simulink model "models_confrontation"  (R2023b)
settings: Solver=VariableStepAuto  StartTime=0.0  StopTime=150  RelTol=1e-3
values from neighbouring files (symbols this model uses):
  A_disc = [0.952255240734 0.0558764138291 0.00101235520744 -0.119343099159 -0.00359337854643 0.0465636781909 0.897600307888 0.0332309130595 0.226714958367 0.0683979085849 0.00118108107535 0.0465232782833 ... (25 elements, 5x5)]    [linear_model.mat]    (also in tank_confrontation_init.m = sys_disc.A)
  B_disc = [0 0 0 0.228023543382 0.0100072301308 0.406395598078 0.00344423879117 -0.350799254632 -0.030419989559 0.036993899484 -0.000142908764649 -0.00850948072699 ... (15 elements, 5x3)]    [linear_model.mat]    (also in tank_confrontation_init.m = sys_disc.B)
  c2_init = c2_0    [tank_confrontation_init.m]
  c3_init = c3_0    [tank_confrontation_init.m]
  C_disc = [0 0 0 1 0 0 0 1 0 0 0 0 ... (15 elements, 3x5)]    [linear_model.mat]    (also in tank_confrontation_init.m = sys_disc.C)
  D_disc = [0  0  0; 0  0  0; 0  0  0]    [linear_model.mat]    (also in tank_confrontation_init.m = sys_disc.D)
  h1_init = h1_0    [tank_confrontation_init.m]
  h2_init = h2_0    [tank_confrontation_init.m]
  h3_init = h3_0    [tank_confrontation_init.m]
  sample_time = 2.0    (= 2)    [tank_confrontation_init.m]
  u_star = [1.78740880431 0.02 0.18]    [linear_model.mat]
  y_star = [x_star(2); x_star(3); x_star(5)]    [tank_confrontation_init.m]
undefined symbols (not defined in the file or in its folder): DiscIntNeverNeededParam, params
libraries: slpidlib x9
settings Model: Creator=fyder9  LastModifiedBy=fyder9

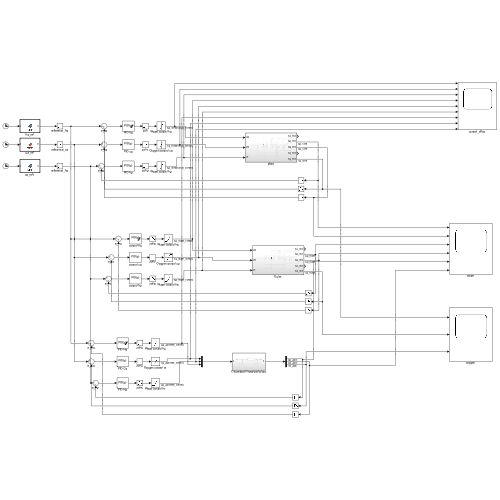
[thumbnail: Simulink's stored preview of the top-level diagram]
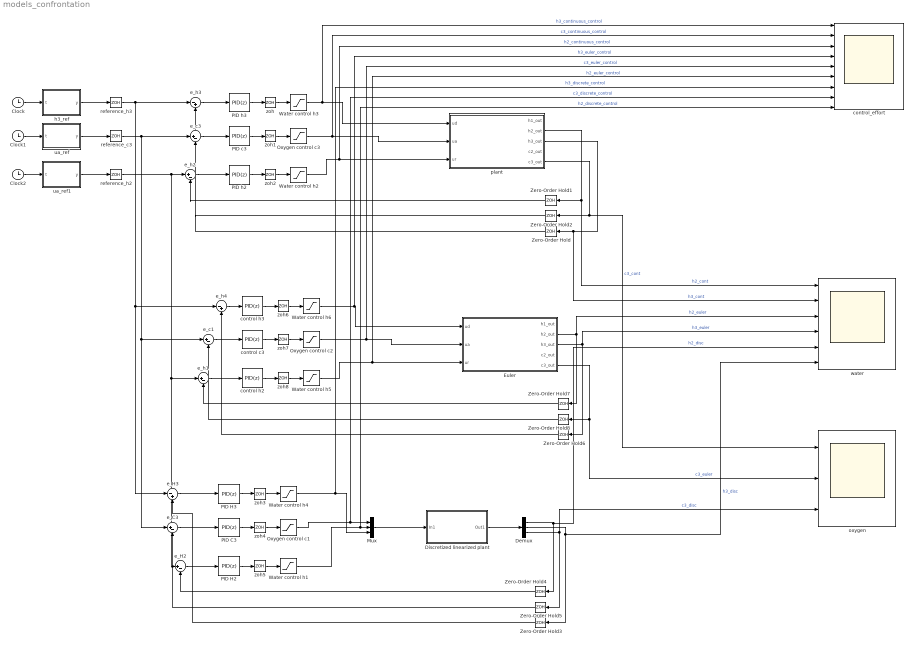
== system models_confrontation ==
  Clock : Clock
  Clock1 : Clock
  Clock2 : Clock
  Demux : Demux  Outputs=3
  Discretized linearized plant : Subsystem
  Euler : Subsystem
  Mux : Mux  Inputs=3
  Oxygen control c1 : Saturate  UpperLimit=1  LowerLimit=0  LinearizeAsGain=off
  Oxygen control c2 : Saturate  UpperLimit=1  LowerLimit=0  LinearizeAsGain=off
  Oxygen control c3 : Saturate  UpperLimit=1  LowerLimit=0  LinearizeAsGain=off
  PID C3 : slpidlib/PID Controller  Controller=PID  Form=Parallel  TimeDomain=Discrete-time  UseExternalTs=off  SampleTime=-1  IntegratorMethod=Forward Euler  FilterMethod=Forward Euler  ControllerParametersSource=internal  P=0.1  I=0.02  UseKiTs=off  D=0  N=100  UseFilter=on  TunerSelectOption=Transfer Function Based (PID Tuner App)  InitialConditionSource=internal  InitialConditionForIntegrator=0  InitialConditionForFilter=0  DifferentiatorICPrevScaledInput=0  ExternalReset=none  TrackingMode=off  Kt=1  LimitOutput=off  SatLimitsSource=internal  UpperSaturationLimit=inf  LowerSaturationLimit=-inf  LinearizeAsGain=off  AntiWindupMode=none  Kb=1  LimitIntegrator=off  UpperIntegratorSaturationLimit=inf  LowerIntegratorSaturationLimit=-inf  POutMin=[]  POutMax=[]  IOutMin=[]  IOutMax=[]  DOutMin=[]  DOutMax=[]  NOutMin=[]  NOutMax=[]  SumOutMin=[]  SumOutMax=[]  SaturationOutMin=[]  SaturationOutMax=[]  PParamMin=[]  PParamMax=[]  IParamMin=[]  IParamMax=[]  DParamMin=[]  DParamMax=[]  NParamMin=[]  NParamMax=[]  KbParamMin=[]  KbParamMax=[]  KtParamMin=[]  KtParamMax=[]  KbOutMin=[]  KbOutMax=[]  KtOutMin=[]  KtOutMax=[]  IntegratorOutMin=[]  IntegratorOutMax=[]  FilterOutMin=[]  FilterOutMax=[]  SumI1OutMin=[]  SumI1OutMax=[]  SumI2OutMin=[]  SumI2OutMax=[]  SumI3OutMin=[]  SumI3OutMax=[]  SumI4OutMin=[]  SumI4OutMax=[]  SumDOutMin=[]  SumDOutMax=[]  DifferentiatorOutMin=[]  DifferentiatorOutMax=[]  FilterDiffOutCoefMin=[]  FilterDiffOutCoefMax=[]  ReciprocalOutMin=[]  ReciprocalOutMax=[]  SumDenOutMin=[]  SumDenOutMax=[]  SumNumOutMin=[]  SumNumOutMax=[]  DivideOutMin=[]  DivideOutMax=[]  UdiffTsProdOutMin=[]  UdiffTsProdOutMax=[]  NTsProdOutMin=[]  NTsProdOutMax=[]  UintegralTsProdOutMin=[]  UintegralTsProdOutMax=[]  UngainTsProdOutMin=[]  UngainTsProdOutMax=[]  ClampingZeroOutDataTypeStr=Inherit: Inherit via back propagation  ClampingZeroOutMin=[]  ClampingZeroOutMax=[]  FilterDenConstantOutDataTypeStr=Inherit: Inherit via back propagation  FilterDenConstantOutMin=[]  FilterDenConstantOutMax=[]  PCopyOutDataTypeStr=Inherit: Inherit via back propagation  PCopyOutMin=[]  PCopyOutMax=[]  NCopyOutDataTypeStr=Inherit: Inherit via back propagation  NCopyOutMin=[]  NCopyOutMax=[]  IntegratorContinuousStateAttributes=''  IntegratorStateMustResolveToSignalObject=off  IntegratorRTWStateStorageClass=Auto  FilterContinuousStateAttributes=''  FilterStateMustResolveToSignalObject=off  FilterRTWStateStorageClass=Auto  ParallelPVariant=InternalParameters  IdealPVariant=Disabled  IVariant=InternalParameters  DVariant=InternalParameters  IntegratorVariant=Discrete  SatVariant=Disabled  AWVariant=Passthrough  PCopyVariant=Disabled  TRVariant=Disabled  FdbkBlocksVariant=Forward  IdealPFdbkVariant=Disabled  SatFdbkVariant=Disabled  DerivativeFilterVariant=ForwardEulerFilter  NVariant=InternalParameters  NCopyVariant=Disabled  FilterICVariant=InternalICsFilter  IntegratorICVariant=InternalICs  ExternalResetVariant=Disabled  TRSumVariant=Passthrough  SumFdbkVariant=Disabled  SumVariant=Sum_PID  TsampFilterVariant=InternalTs  TsampNgainVariant=Passthrough  TsampIntegralVariant=Disabled_SignalSpec  ExternalSaturationOutDataTypeStr=Inherit: Same as second input
      settings: LibrarySourceBlock=simulink/Discrete/Discrete PID Controller
  PID H2 : slpidlib/PID Controller  Controller=PID  Form=Parallel  TimeDomain=Discrete-time  UseExternalTs=off  SampleTime=-1  IntegratorMethod=Forward Euler  FilterMethod=Forward Euler  ControllerParametersSource=internal  P=0.2  I=0.03  UseKiTs=off  D=0  N=100  UseFilter=on  TunerSelectOption=Transfer Function Based (PID Tuner App)  InitialConditionSource=internal  InitialConditionForIntegrator=0  InitialConditionForFilter=0  DifferentiatorICPrevScaledInput=0  ExternalReset=none  TrackingMode=off  Kt=1  LimitOutput=off  SatLimitsSource=internal  UpperSaturationLimit=inf  LowerSaturationLimit=-inf  LinearizeAsGain=off  AntiWindupMode=none  Kb=1  LimitIntegrator=off  UpperIntegratorSaturationLimit=inf  LowerIntegratorSaturationLimit=-inf  POutMin=[]  POutMax=[]  IOutMin=[]  IOutMax=[]  DOutMin=[]  DOutMax=[]  NOutMin=[]  NOutMax=[]  SumOutMin=[]  SumOutMax=[]  SaturationOutMin=[]  SaturationOutMax=[]  PParamMin=[]  PParamMax=[]  IParamMin=[]  IParamMax=[]  DParamMin=[]  DParamMax=[]  NParamMin=[]  NParamMax=[]  KbParamMin=[]  KbParamMax=[]  KtParamMin=[]  KtParamMax=[]  KbOutMin=[]  KbOutMax=[]  KtOutMin=[]  KtOutMax=[]  IntegratorOutMin=[]  IntegratorOutMax=[]  FilterOutMin=[]  FilterOutMax=[]  SumI1OutMin=[]  SumI1OutMax=[]  SumI2OutMin=[]  SumI2OutMax=[]  SumI3OutMin=[]  SumI3OutMax=[]  SumI4OutMin=[]  SumI4OutMax=[]  SumDOutMin=[]  SumDOutMax=[]  DifferentiatorOutMin=[]  DifferentiatorOutMax=[]  FilterDiffOutCoefMin=[]  FilterDiffOutCoefMax=[]  ReciprocalOutMin=[]  ReciprocalOutMax=[]  SumDenOutMin=[]  SumDenOutMax=[]  SumNumOutMin=[]  SumNumOutMax=[]  DivideOutMin=[]  DivideOutMax=[]  UdiffTsProdOutMin=[]  UdiffTsProdOutMax=[]  NTsProdOutMin=[]  NTsProdOutMax=[]  UintegralTsProdOutMin=[]  UintegralTsProdOutMax=[]  UngainTsProdOutMin=[]  UngainTsProdOutMax=[]  ClampingZeroOutDataTypeStr=Inherit: Inherit via back propagation  ClampingZeroOutMin=[]  ClampingZeroOutMax=[]  FilterDenConstantOutDataTypeStr=Inherit: Inherit via back propagation  FilterDenConstantOutMin=[]  FilterDenConstantOutMax=[]  PCopyOutDataTypeStr=Inherit: Inherit via back propagation  PCopyOutMin=[]  PCopyOutMax=[]  NCopyOutDataTypeStr=Inherit: Inherit via back propagation  NCopyOutMin=[]  NCopyOutMax=[]  IntegratorContinuousStateAttributes=''  IntegratorStateMustResolveToSignalObject=off  IntegratorRTWStateStorageClass=Auto  FilterContinuousStateAttributes=''  FilterStateMustResolveToSignalObject=off  FilterRTWStateStorageClass=Auto  ParallelPVariant=InternalParameters  IdealPVariant=Disabled  IVariant=InternalParameters  DVariant=InternalParameters  IntegratorVariant=Discrete  SatVariant=Disabled  AWVariant=Passthrough  PCopyVariant=Disabled  TRVariant=Disabled  FdbkBlocksVariant=Forward  IdealPFdbkVariant=Disabled  SatFdbkVariant=Disabled  DerivativeFilterVariant=ForwardEulerFilter  NVariant=InternalParameters  NCopyVariant=Disabled  FilterICVariant=InternalICsFilter  IntegratorICVariant=InternalICs  ExternalResetVariant=Disabled  TRSumVariant=Passthrough  SumFdbkVariant=Disabled  SumVariant=Sum_PID  TsampFilterVariant=InternalTs  TsampNgainVariant=Passthrough  TsampIntegralVariant=Disabled_SignalSpec  ExternalSaturationOutDataTypeStr=Inherit: Same as second input
      settings: LibrarySourceBlock=simulink/Discrete/Discrete PID Controller
  PID H3 : slpidlib/PID Controller  Controller=PID  Form=Parallel  TimeDomain=Discrete-time  UseExternalTs=off  SampleTime=-1  IntegratorMethod=Forward Euler  FilterMethod=Forward Euler  ControllerParametersSource=internal  P=0.6  I=0.08  UseKiTs=off  D=0  N=100  UseFilter=on  TunerSelectOption=Transfer Function Based (PID Tuner App)  InitialConditionSource=internal  InitialConditionForIntegrator=0  InitialConditionForFilter=0  DifferentiatorICPrevScaledInput=0  ExternalReset=none  TrackingMode=off  Kt=1  LimitOutput=on  SatLimitsSource=internal  UpperSaturationLimit=inf  LowerSaturationLimit=-inf  LinearizeAsGain=off  AntiWindupMode=clamping  Kb=1  LimitIntegrator=off  UpperIntegratorSaturationLimit=inf  LowerIntegratorSaturationLimit=-inf  POutMin=[]  POutMax=[]  IOutMin=[]  IOutMax=[]  DOutMin=[]  DOutMax=[]  NOutMin=[]  NOutMax=[]  SumOutMin=[]  SumOutMax=[]  SaturationOutMin=[]  SaturationOutMax=[]  PParamMin=[]  PParamMax=[]  IParamMin=[]  IParamMax=[]  DParamMin=[]  DParamMax=[]  NParamMin=[]  NParamMax=[]  KbParamMin=[]  KbParamMax=[]  KtParamMin=[]  KtParamMax=[]  KbOutMin=[]  KbOutMax=[]  KtOutMin=[]  KtOutMax=[]  IntegratorOutMin=[]  IntegratorOutMax=[]  FilterOutMin=[]  FilterOutMax=[]  SumI1OutMin=[]  SumI1OutMax=[]  SumI2OutMin=[]  SumI2OutMax=[]  SumI3OutMin=[]  SumI3OutMax=[]  SumI4OutMin=[]  SumI4OutMax=[]  SumDOutMin=[]  SumDOutMax=[]  DifferentiatorOutMin=[]  DifferentiatorOutMax=[]  FilterDiffOutCoefMin=[]  FilterDiffOutCoefMax=[]  ReciprocalOutMin=[]  ReciprocalOutMax=[]  SumDenOutMin=[]  SumDenOutMax=[]  SumNumOutMin=[]  SumNumOutMax=[]  DivideOutMin=[]  DivideOutMax=[]  UdiffTsProdOutMin=[]  UdiffTsProdOutMax=[]  NTsProdOutMin=[]  NTsProdOutMax=[]  UintegralTsProdOutMin=[]  UintegralTsProdOutMax=[]  UngainTsProdOutMin=[]  UngainTsProdOutMax=[]  ClampingZeroOutDataTypeStr=Inherit: Inherit via back propagation  ClampingZeroOutMin=[]  ClampingZeroOutMax=[]  FilterDenConstantOutDataTypeStr=Inherit: Inherit via back propagation  FilterDenConstantOutMin=[]  FilterDenConstantOutMax=[]  PCopyOutDataTypeStr=Inherit: Inherit via back propagation  PCopyOutMin=[]  PCopyOutMax=[]  NCopyOutDataTypeStr=Inherit: Inherit via back propagation  NCopyOutMin=[]  NCopyOutMax=[]  IntegratorContinuousStateAttributes=''  IntegratorStateMustResolveToSignalObject=off  IntegratorRTWStateStorageClass=Auto  FilterContinuousStateAttributes=''  FilterStateMustResolveToSignalObject=off  FilterRTWStateStorageClass=Auto  ParallelPVariant=InternalParameters  IdealPVariant=Disabled  IVariant=InternalParameters  DVariant=InternalParameters  IntegratorVariant=Discrete  SatVariant=Enabled  AWVariant=DiscClampingParallel  PCopyVariant=Disabled  TRVariant=Disabled  FdbkBlocksVariant=Forward  IdealPFdbkVariant=Disabled  SatFdbkVariant=Disabled  DerivativeFilterVariant=ForwardEulerFilter  NVariant=InternalParameters  NCopyVariant=Disabled  FilterICVariant=InternalICsFilter  IntegratorICVariant=InternalICs  ExternalResetVariant=Disabled  TRSumVariant=Passthrough  SumFdbkVariant=Disabled  SumVariant=Sum_PID  TsampFilterVariant=InternalTs  TsampNgainVariant=Passthrough  TsampIntegralVariant=Disabled_SignalSpec  ExternalSaturationOutDataTypeStr=Inherit: Same as second input
      settings: LibrarySourceBlock=simulink/Discrete/Discrete PID Controller
  PID c3 : slpidlib/PID Controller  Controller=PID  Form=Parallel  TimeDomain=Discrete-time  UseExternalTs=off  SampleTime=-1  IntegratorMethod=Forward Euler  FilterMethod=Forward Euler  ControllerParametersSource=internal  P=0.1  I=0.02  UseKiTs=off  D=0  N=100  UseFilter=on  TunerSelectOption=Transfer Function Based (PID Tuner App)  InitialConditionSource=internal  InitialConditionForIntegrator=0  InitialConditionForFilter=0  DifferentiatorICPrevScaledInput=0  ExternalReset=none  TrackingMode=off  Kt=1  LimitOutput=off  SatLimitsSource=internal  UpperSaturationLimit=inf  LowerSaturationLimit=-inf  LinearizeAsGain=off  AntiWindupMode=none  Kb=1  LimitIntegrator=off  UpperIntegratorSaturationLimit=inf  LowerIntegratorSaturationLimit=-inf  POutMin=[]  POutMax=[]  IOutMin=[]  IOutMax=[]  DOutMin=[]  DOutMax=[]  NOutMin=[]  NOutMax=[]  SumOutMin=[]  SumOutMax=[]  SaturationOutMin=[]  SaturationOutMax=[]  PParamMin=[]  PParamMax=[]  IParamMin=[]  IParamMax=[]  DParamMin=[]  DParamMax=[]  NParamMin=[]  NParamMax=[]  KbParamMin=[]  KbParamMax=[]  KtParamMin=[]  KtParamMax=[]  KbOutMin=[]  KbOutMax=[]  KtOutMin=[]  KtOutMax=[]  IntegratorOutMin=[]  IntegratorOutMax=[]  FilterOutMin=[]  FilterOutMax=[]  SumI1OutMin=[]  SumI1OutMax=[]  SumI2OutMin=[]  SumI2OutMax=[]  SumI3OutMin=[]  SumI3OutMax=[]  SumI4OutMin=[]  SumI4OutMax=[]  SumDOutMin=[]  SumDOutMax=[]  DifferentiatorOutMin=[]  DifferentiatorOutMax=[]  FilterDiffOutCoefMin=[]  FilterDiffOutCoefMax=[]  ReciprocalOutMin=[]  ReciprocalOutMax=[]  SumDenOutMin=[]  SumDenOutMax=[]  SumNumOutMin=[]  SumNumOutMax=[]  DivideOutMin=[]  DivideOutMax=[]  UdiffTsProdOutMin=[]  UdiffTsProdOutMax=[]  NTsProdOutMin=[]  NTsProdOutMax=[]  UintegralTsProdOutMin=[]  UintegralTsProdOutMax=[]  UngainTsProdOutMin=[]  UngainTsProdOutMax=[]  ClampingZeroOutDataTypeStr=Inherit: Inherit via back propagation  ClampingZeroOutMin=[]  ClampingZeroOutMax=[]  FilterDenConstantOutDataTypeStr=Inherit: Inherit via back propagation  FilterDenConstantOutMin=[]  FilterDenConstantOutMax=[]  PCopyOutDataTypeStr=Inherit: Inherit via back propagation  PCopyOutMin=[]  PCopyOutMax=[]  NCopyOutDataTypeStr=Inherit: Inherit via back propagation  NCopyOutMin=[]  NCopyOutMax=[]  IntegratorContinuousStateAttributes=''  IntegratorStateMustResolveToSignalObject=off  IntegratorRTWStateStorageClass=Auto  FilterContinuousStateAttributes=''  FilterStateMustResolveToSignalObject=off  FilterRTWStateStorageClass=Auto  ParallelPVariant=InternalParameters  IdealPVariant=Disabled  IVariant=InternalParameters  DVariant=InternalParameters  IntegratorVariant=Discrete  SatVariant=Disabled  AWVariant=Passthrough  PCopyVariant=Disabled  TRVariant=Disabled  FdbkBlocksVariant=Forward  IdealPFdbkVariant=Disabled  SatFdbkVariant=Disabled  DerivativeFilterVariant=ForwardEulerFilter  NVariant=InternalParameters  NCopyVariant=Disabled  FilterICVariant=InternalICsFilter  IntegratorICVariant=InternalICs  ExternalResetVariant=Disabled  TRSumVariant=Passthrough  SumFdbkVariant=Disabled  SumVariant=Sum_PID  TsampFilterVariant=InternalTs  TsampNgainVariant=Passthrough  TsampIntegralVariant=Disabled_SignalSpec  ExternalSaturationOutDataTypeStr=Inherit: Same as second input
      settings: LibrarySourceBlock=simulink/Discrete/Discrete PID Controller
  PID h2 : slpidlib/PID Controller  Controller=PID  Form=Parallel  TimeDomain=Discrete-time  UseExternalTs=off  SampleTime=-1  IntegratorMethod=Forward Euler  FilterMethod=Forward Euler  ControllerParametersSource=internal  P=0.2  I=0.03  UseKiTs=off  D=0  N=100  UseFilter=on  TunerSelectOption=Transfer Function Based (PID Tuner App)  InitialConditionSource=internal  InitialConditionForIntegrator=0  InitialConditionForFilter=0  DifferentiatorICPrevScaledInput=0  ExternalReset=none  TrackingMode=off  Kt=1  LimitOutput=off  SatLimitsSource=internal  UpperSaturationLimit=inf  LowerSaturationLimit=-inf  LinearizeAsGain=off  AntiWindupMode=none  Kb=1  LimitIntegrator=off  UpperIntegratorSaturationLimit=inf  LowerIntegratorSaturationLimit=-inf  POutMin=[]  POutMax=[]  IOutMin=[]  IOutMax=[]  DOutMin=[]  DOutMax=[]  NOutMin=[]  NOutMax=[]  SumOutMin=[]  SumOutMax=[]  SaturationOutMin=[]  SaturationOutMax=[]  PParamMin=[]  PParamMax=[]  IParamMin=[]  IParamMax=[]  DParamMin=[]  DParamMax=[]  NParamMin=[]  NParamMax=[]  KbParamMin=[]  KbParamMax=[]  KtParamMin=[]  KtParamMax=[]  KbOutMin=[]  KbOutMax=[]  KtOutMin=[]  KtOutMax=[]  IntegratorOutMin=[]  IntegratorOutMax=[]  FilterOutMin=[]  FilterOutMax=[]  SumI1OutMin=[]  SumI1OutMax=[]  SumI2OutMin=[]  SumI2OutMax=[]  SumI3OutMin=[]  SumI3OutMax=[]  SumI4OutMin=[]  SumI4OutMax=[]  SumDOutMin=[]  SumDOutMax=[]  DifferentiatorOutMin=[]  DifferentiatorOutMax=[]  FilterDiffOutCoefMin=[]  FilterDiffOutCoefMax=[]  ReciprocalOutMin=[]  ReciprocalOutMax=[]  SumDenOutMin=[]  SumDenOutMax=[]  SumNumOutMin=[]  SumNumOutMax=[]  DivideOutMin=[]  DivideOutMax=[]  UdiffTsProdOutMin=[]  UdiffTsProdOutMax=[]  NTsProdOutMin=[]  NTsProdOutMax=[]  UintegralTsProdOutMin=[]  UintegralTsProdOutMax=[]  UngainTsProdOutMin=[]  UngainTsProdOutMax=[]  ClampingZeroOutDataTypeStr=Inherit: Inherit via back propagation  ClampingZeroOutMin=[]  ClampingZeroOutMax=[]  FilterDenConstantOutDataTypeStr=Inherit: Inherit via back propagation  FilterDenConstantOutMin=[]  FilterDenConstantOutMax=[]  PCopyOutDataTypeStr=Inherit: Inherit via back propagation  PCopyOutMin=[]  PCopyOutMax=[]  NCopyOutDataTypeStr=Inherit: Inherit via back propagation  NCopyOutMin=[]  NCopyOutMax=[]  IntegratorContinuousStateAttributes=''  IntegratorStateMustResolveToSignalObject=off  IntegratorRTWStateStorageClass=Auto  FilterContinuousStateAttributes=''  FilterStateMustResolveToSignalObject=off  FilterRTWStateStorageClass=Auto  ParallelPVariant=InternalParameters  IdealPVariant=Disabled  IVariant=InternalParameters  DVariant=InternalParameters  IntegratorVariant=Discrete  SatVariant=Disabled  AWVariant=Passthrough  PCopyVariant=Disabled  TRVariant=Disabled  FdbkBlocksVariant=Forward  IdealPFdbkVariant=Disabled  SatFdbkVariant=Disabled  DerivativeFilterVariant=ForwardEulerFilter  NVariant=InternalParameters  NCopyVariant=Disabled  FilterICVariant=InternalICsFilter  IntegratorICVariant=InternalICs  ExternalResetVariant=Disabled  TRSumVariant=Passthrough  SumFdbkVariant=Disabled  SumVariant=Sum_PID  TsampFilterVariant=InternalTs  TsampNgainVariant=Passthrough  TsampIntegralVariant=Disabled_SignalSpec  ExternalSaturationOutDataTypeStr=Inherit: Same as second input
      settings: LibrarySourceBlock=simulink/Discrete/Discrete PID Controller
  PID h3 : slpidlib/PID Controller  Controller=PID  Form=Parallel  TimeDomain=Discrete-time  UseExternalTs=off  SampleTime=-1  IntegratorMethod=Forward Euler  FilterMethod=Forward Euler  ControllerParametersSource=internal  P=0.6  I=0.08  UseKiTs=off  D=0  N=100  UseFilter=on  TunerSelectOption=Transfer Function Based (PID Tuner App)  InitialConditionSource=internal  InitialConditionForIntegrator=0  InitialConditionForFilter=0  DifferentiatorICPrevScaledInput=0  ExternalReset=none  TrackingMode=off  Kt=1  LimitOutput=on  SatLimitsSource=internal  UpperSaturationLimit=inf  LowerSaturationLimit=-inf  LinearizeAsGain=off  AntiWindupMode=clamping  Kb=1  LimitIntegrator=off  UpperIntegratorSaturationLimit=inf  LowerIntegratorSaturationLimit=-inf  POutMin=[]  POutMax=[]  IOutMin=[]  IOutMax=[]  DOutMin=[]  DOutMax=[]  NOutMin=[]  NOutMax=[]  SumOutMin=[]  SumOutMax=[]  SaturationOutMin=[]  SaturationOutMax=[]  PParamMin=[]  PParamMax=[]  IParamMin=[]  IParamMax=[]  DParamMin=[]  DParamMax=[]  NParamMin=[]  NParamMax=[]  KbParamMin=[]  KbParamMax=[]  KtParamMin=[]  KtParamMax=[]  KbOutMin=[]  KbOutMax=[]  KtOutMin=[]  KtOutMax=[]  IntegratorOutMin=[]  IntegratorOutMax=[]  FilterOutMin=[]  FilterOutMax=[]  SumI1OutMin=[]  SumI1OutMax=[]  SumI2OutMin=[]  SumI2OutMax=[]  SumI3OutMin=[]  SumI3OutMax=[]  SumI4OutMin=[]  SumI4OutMax=[]  SumDOutMin=[]  SumDOutMax=[]  DifferentiatorOutMin=[]  DifferentiatorOutMax=[]  FilterDiffOutCoefMin=[]  FilterDiffOutCoefMax=[]  ReciprocalOutMin=[]  ReciprocalOutMax=[]  SumDenOutMin=[]  SumDenOutMax=[]  SumNumOutMin=[]  SumNumOutMax=[]  DivideOutMin=[]  DivideOutMax=[]  UdiffTsProdOutMin=[]  UdiffTsProdOutMax=[]  NTsProdOutMin=[]  NTsProdOutMax=[]  UintegralTsProdOutMin=[]  UintegralTsProdOutMax=[]  UngainTsProdOutMin=[]  UngainTsProdOutMax=[]  ClampingZeroOutDataTypeStr=Inherit: Inherit via back propagation  ClampingZeroOutMin=[]  ClampingZeroOutMax=[]  FilterDenConstantOutDataTypeStr=Inherit: Inherit via back propagation  FilterDenConstantOutMin=[]  FilterDenConstantOutMax=[]  PCopyOutDataTypeStr=Inherit: Inherit via back propagation  PCopyOutMin=[]  PCopyOutMax=[]  NCopyOutDataTypeStr=Inherit: Inherit via back propagation  NCopyOutMin=[]  NCopyOutMax=[]  IntegratorContinuousStateAttributes=''  IntegratorStateMustResolveToSignalObject=off  IntegratorRTWStateStorageClass=Auto  FilterContinuousStateAttributes=''  FilterStateMustResolveToSignalObject=off  FilterRTWStateStorageClass=Auto  ParallelPVariant=InternalParameters  IdealPVariant=Disabled  IVariant=InternalParameters  DVariant=InternalParameters  IntegratorVariant=Discrete  SatVariant=Enabled  AWVariant=DiscClampingParallel  PCopyVariant=Disabled  TRVariant=Disabled  FdbkBlocksVariant=Forward  IdealPFdbkVariant=Disabled  SatFdbkVariant=Disabled  DerivativeFilterVariant=ForwardEulerFilter  NVariant=InternalParameters  NCopyVariant=Disabled  FilterICVariant=InternalICsFilter  IntegratorICVariant=InternalICs  ExternalResetVariant=Disabled  TRSumVariant=Passthrough  SumFdbkVariant=Disabled  SumVariant=Sum_PID  TsampFilterVariant=InternalTs  TsampNgainVariant=Passthrough  TsampIntegralVariant=Disabled_SignalSpec  ExternalSaturationOutDataTypeStr=Inherit: Same as second input
      settings: LibrarySourceBlock=simulink/Discrete/Discrete PID Controller
  Water control h{1..6} (6 alike) : Saturate  UpperLimit=0.25  LowerLimit=0.05  LinearizeAsGain=off
  Zero-Order Hold{,1..8} (9 alike) : ZeroOrderHold  SampleTime=sample_time
  control c3 : slpidlib/PID Controller  Controller=PID  Form=Parallel  TimeDomain=Discrete-time  UseExternalTs=off  SampleTime=-1  IntegratorMethod=Forward Euler  FilterMethod=Forward Euler  ControllerParametersSource=internal  P=0.1  I=0.02  UseKiTs=off  D=0  N=100  UseFilter=on  TunerSelectOption=Transfer Function Based (PID Tuner App)  InitialConditionSource=internal  InitialConditionForIntegrator=0  InitialConditionForFilter=0  DifferentiatorICPrevScaledInput=0  ExternalReset=none  TrackingMode=off  Kt=1  LimitOutput=off  SatLimitsSource=internal  UpperSaturationLimit=inf  LowerSaturationLimit=-inf  LinearizeAsGain=off  AntiWindupMode=none  Kb=1  LimitIntegrator=off  UpperIntegratorSaturationLimit=inf  LowerIntegratorSaturationLimit=-inf  POutMin=[]  POutMax=[]  IOutMin=[]  IOutMax=[]  DOutMin=[]  DOutMax=[]  NOutMin=[]  NOutMax=[]  SumOutMin=[]  SumOutMax=[]  SaturationOutMin=[]  SaturationOutMax=[]  PParamMin=[]  PParamMax=[]  IParamMin=[]  IParamMax=[]  DParamMin=[]  DParamMax=[]  NParamMin=[]  NParamMax=[]  KbParamMin=[]  KbParamMax=[]  KtParamMin=[]  KtParamMax=[]  KbOutMin=[]  KbOutMax=[]  KtOutMin=[]  KtOutMax=[]  IntegratorOutMin=[]  IntegratorOutMax=[]  FilterOutMin=[]  FilterOutMax=[]  SumI1OutMin=[]  SumI1OutMax=[]  SumI2OutMin=[]  SumI2OutMax=[]  SumI3OutMin=[]  SumI3OutMax=[]  SumI4OutMin=[]  SumI4OutMax=[]  SumDOutMin=[]  SumDOutMax=[]  DifferentiatorOutMin=[]  DifferentiatorOutMax=[]  FilterDiffOutCoefMin=[]  FilterDiffOutCoefMax=[]  ReciprocalOutMin=[]  ReciprocalOutMax=[]  SumDenOutMin=[]  SumDenOutMax=[]  SumNumOutMin=[]  SumNumOutMax=[]  DivideOutMin=[]  DivideOutMax=[]  UdiffTsProdOutMin=[]  UdiffTsProdOutMax=[]  NTsProdOutMin=[]  NTsProdOutMax=[]  UintegralTsProdOutMin=[]  UintegralTsProdOutMax=[]  UngainTsProdOutMin=[]  UngainTsProdOutMax=[]  ClampingZeroOutDataTypeStr=Inherit: Inherit via back propagation  ClampingZeroOutMin=[]  ClampingZeroOutMax=[]  FilterDenConstantOutDataTypeStr=Inherit: Inherit via back propagation  FilterDenConstantOutMin=[]  FilterDenConstantOutMax=[]  PCopyOutDataTypeStr=Inherit: Inherit via back propagation  PCopyOutMin=[]  PCopyOutMax=[]  NCopyOutDataTypeStr=Inherit: Inherit via back propagation  NCopyOutMin=[]  NCopyOutMax=[]  IntegratorContinuousStateAttributes=''  IntegratorStateMustResolveToSignalObject=off  IntegratorRTWStateStorageClass=Auto  FilterContinuousStateAttributes=''  FilterStateMustResolveToSignalObject=off  FilterRTWStateStorageClass=Auto  ParallelPVariant=InternalParameters  IdealPVariant=Disabled  IVariant=InternalParameters  DVariant=InternalParameters  IntegratorVariant=Discrete  SatVariant=Disabled  AWVariant=Passthrough  PCopyVariant=Disabled  TRVariant=Disabled  FdbkBlocksVariant=Forward  IdealPFdbkVariant=Disabled  SatFdbkVariant=Disabled  DerivativeFilterVariant=ForwardEulerFilter  NVariant=InternalParameters  NCopyVariant=Disabled  FilterICVariant=InternalICsFilter  IntegratorICVariant=InternalICs  ExternalResetVariant=Disabled  TRSumVariant=Passthrough  SumFdbkVariant=Disabled  SumVariant=Sum_PID  TsampFilterVariant=InternalTs  TsampNgainVariant=Passthrough  TsampIntegralVariant=Disabled_SignalSpec  ExternalSaturationOutDataTypeStr=Inherit: Same as second input
      settings: LibrarySourceBlock=simulink/Discrete/Discrete PID Controller
  control h2 : slpidlib/PID Controller  Controller=PID  Form=Parallel  TimeDomain=Discrete-time  UseExternalTs=off  SampleTime=-1  IntegratorMethod=Forward Euler  FilterMethod=Forward Euler  ControllerParametersSource=internal  P=0.2  I=0.03  UseKiTs=off  D=0  N=100  UseFilter=on  TunerSelectOption=Transfer Function Based (PID Tuner App)  InitialConditionSource=internal  InitialConditionForIntegrator=0  InitialConditionForFilter=0  DifferentiatorICPrevScaledInput=0  ExternalReset=none  TrackingMode=off  Kt=1  LimitOutput=off  SatLimitsSource=internal  UpperSaturationLimit=inf  LowerSaturationLimit=-inf  LinearizeAsGain=off  AntiWindupMode=none  Kb=1  LimitIntegrator=off  UpperIntegratorSaturationLimit=inf  LowerIntegratorSaturationLimit=-inf  POutMin=[]  POutMax=[]  IOutMin=[]  IOutMax=[]  DOutMin=[]  DOutMax=[]  NOutMin=[]  NOutMax=[]  SumOutMin=[]  SumOutMax=[]  SaturationOutMin=[]  SaturationOutMax=[]  PParamMin=[]  PParamMax=[]  IParamMin=[]  IParamMax=[]  DParamMin=[]  DParamMax=[]  NParamMin=[]  NParamMax=[]  KbParamMin=[]  KbParamMax=[]  KtParamMin=[]  KtParamMax=[]  KbOutMin=[]  KbOutMax=[]  KtOutMin=[]  KtOutMax=[]  IntegratorOutMin=[]  IntegratorOutMax=[]  FilterOutMin=[]  FilterOutMax=[]  SumI1OutMin=[]  SumI1OutMax=[]  SumI2OutMin=[]  SumI2OutMax=[]  SumI3OutMin=[]  SumI3OutMax=[]  SumI4OutMin=[]  SumI4OutMax=[]  SumDOutMin=[]  SumDOutMax=[]  DifferentiatorOutMin=[]  DifferentiatorOutMax=[]  FilterDiffOutCoefMin=[]  FilterDiffOutCoefMax=[]  ReciprocalOutMin=[]  ReciprocalOutMax=[]  SumDenOutMin=[]  SumDenOutMax=[]  SumNumOutMin=[]  SumNumOutMax=[]  DivideOutMin=[]  DivideOutMax=[]  UdiffTsProdOutMin=[]  UdiffTsProdOutMax=[]  NTsProdOutMin=[]  NTsProdOutMax=[]  UintegralTsProdOutMin=[]  UintegralTsProdOutMax=[]  UngainTsProdOutMin=[]  UngainTsProdOutMax=[]  ClampingZeroOutDataTypeStr=Inherit: Inherit via back propagation  ClampingZeroOutMin=[]  ClampingZeroOutMax=[]  FilterDenConstantOutDataTypeStr=Inherit: Inherit via back propagation  FilterDenConstantOutMin=[]  FilterDenConstantOutMax=[]  PCopyOutDataTypeStr=Inherit: Inherit via back propagation  PCopyOutMin=[]  PCopyOutMax=[]  NCopyOutDataTypeStr=Inherit: Inherit via back propagation  NCopyOutMin=[]  NCopyOutMax=[]  IntegratorContinuousStateAttributes=''  IntegratorStateMustResolveToSignalObject=off  IntegratorRTWStateStorageClass=Auto  FilterContinuousStateAttributes=''  FilterStateMustResolveToSignalObject=off  FilterRTWStateStorageClass=Auto  ParallelPVariant=InternalParameters  IdealPVariant=Disabled  IVariant=InternalParameters  DVariant=InternalParameters  IntegratorVariant=Discrete  SatVariant=Disabled  AWVariant=Passthrough  PCopyVariant=Disabled  TRVariant=Disabled  FdbkBlocksVariant=Forward  IdealPFdbkVariant=Disabled  SatFdbkVariant=Disabled  DerivativeFilterVariant=ForwardEulerFilter  NVariant=InternalParameters  NCopyVariant=Disabled  FilterICVariant=InternalICsFilter  IntegratorICVariant=InternalICs  ExternalResetVariant=Disabled  TRSumVariant=Passthrough  SumFdbkVariant=Disabled  SumVariant=Sum_PID  TsampFilterVariant=InternalTs  TsampNgainVariant=Passthrough  TsampIntegralVariant=Disabled_SignalSpec  ExternalSaturationOutDataTypeStr=Inherit: Same as second input
      settings: LibrarySourceBlock=simulink/Discrete/Discrete PID Controller
  control h3 : slpidlib/PID Controller  Controller=PID  Form=Parallel  TimeDomain=Discrete-time  UseExternalTs=off  SampleTime=-1  IntegratorMethod=Forward Euler  FilterMethod=Forward Euler  ControllerParametersSource=internal  P=0.6  I=0.08  UseKiTs=off  D=0  N=100  UseFilter=on  TunerSelectOption=Transfer Function Based (PID Tuner App)  InitialConditionSource=internal  InitialConditionForIntegrator=0  InitialConditionForFilter=0  DifferentiatorICPrevScaledInput=0  ExternalReset=none  TrackingMode=off  Kt=1  LimitOutput=on  SatLimitsSource=internal  UpperSaturationLimit=inf  LowerSaturationLimit=-inf  LinearizeAsGain=off  AntiWindupMode=clamping  Kb=1  LimitIntegrator=off  UpperIntegratorSaturationLimit=inf  LowerIntegratorSaturationLimit=-inf  POutMin=[]  POutMax=[]  IOutMin=[]  IOutMax=[]  DOutMin=[]  DOutMax=[]  NOutMin=[]  NOutMax=[]  SumOutMin=[]  SumOutMax=[]  SaturationOutMin=[]  SaturationOutMax=[]  PParamMin=[]  PParamMax=[]  IParamMin=[]  IParamMax=[]  DParamMin=[]  DParamMax=[]  NParamMin=[]  NParamMax=[]  KbParamMin=[]  KbParamMax=[]  KtParamMin=[]  KtParamMax=[]  KbOutMin=[]  KbOutMax=[]  KtOutMin=[]  KtOutMax=[]  IntegratorOutMin=[]  IntegratorOutMax=[]  FilterOutMin=[]  FilterOutMax=[]  SumI1OutMin=[]  SumI1OutMax=[]  SumI2OutMin=[]  SumI2OutMax=[]  SumI3OutMin=[]  SumI3OutMax=[]  SumI4OutMin=[]  SumI4OutMax=[]  SumDOutMin=[]  SumDOutMax=[]  DifferentiatorOutMin=[]  DifferentiatorOutMax=[]  FilterDiffOutCoefMin=[]  FilterDiffOutCoefMax=[]  ReciprocalOutMin=[]  ReciprocalOutMax=[]  SumDenOutMin=[]  SumDenOutMax=[]  SumNumOutMin=[]  SumNumOutMax=[]  DivideOutMin=[]  DivideOutMax=[]  UdiffTsProdOutMin=[]  UdiffTsProdOutMax=[]  NTsProdOutMin=[]  NTsProdOutMax=[]  UintegralTsProdOutMin=[]  UintegralTsProdOutMax=[]  UngainTsProdOutMin=[]  UngainTsProdOutMax=[]  ClampingZeroOutDataTypeStr=Inherit: Inherit via back propagation  ClampingZeroOutMin=[]  ClampingZeroOutMax=[]  FilterDenConstantOutDataTypeStr=Inherit: Inherit via back propagation  FilterDenConstantOutMin=[]  FilterDenConstantOutMax=[]  PCopyOutDataTypeStr=Inherit: Inherit via back propagation  PCopyOutMin=[]  PCopyOutMax=[]  NCopyOutDataTypeStr=Inherit: Inherit via back propagation  NCopyOutMin=[]  NCopyOutMax=[]  IntegratorContinuousStateAttributes=''  IntegratorStateMustResolveToSignalObject=off  IntegratorRTWStateStorageClass=Auto  FilterContinuousStateAttributes=''  FilterStateMustResolveToSignalObject=off  FilterRTWStateStorageClass=Auto  ParallelPVariant=InternalParameters  IdealPVariant=Disabled  IVariant=InternalParameters  DVariant=InternalParameters  IntegratorVariant=Discrete  SatVariant=Enabled  AWVariant=DiscClampingParallel  PCopyVariant=Disabled  TRVariant=Disabled  FdbkBlocksVariant=Forward  IdealPFdbkVariant=Disabled  SatFdbkVariant=Disabled  DerivativeFilterVariant=ForwardEulerFilter  NVariant=InternalParameters  NCopyVariant=Disabled  FilterICVariant=InternalICsFilter  IntegratorICVariant=InternalICs  ExternalResetVariant=Disabled  TRSumVariant=Passthrough  SumFdbkVariant=Disabled  SumVariant=Sum_PID  TsampFilterVariant=InternalTs  TsampNgainVariant=Passthrough  TsampIntegralVariant=Disabled_SignalSpec  ExternalSaturationOutDataTypeStr=Inherit: Same as second input
      settings: LibrarySourceBlock=simulink/Discrete/Discrete PID Controller
  control_effort : Scope  NumInputPorts=9
  e_C3 : Sum  Inputs=|+-
  e_H2 : Sum  Inputs=|+-
  e_H3 : Sum  Inputs=|-+
  e_c1 : Sum  Inputs=|+-
  e_c3 : Sum  Inputs=|+-
  e_h1 : Sum  Inputs=|+-
  e_h2 : Sum  Inputs=|+-
  e_h3 : Sum  Inputs=|-+
  e_h4 : Sum  Inputs=|-+
  h3_ref : MATLAB Function  TreatAsAtomicUnit=on
  oxygen : Scope  NumInputPorts=3
  plant : Subsystem
  reference_c3 : ZeroOrderHold  SampleTime=sample_time
  reference_h2 : ZeroOrderHold  SampleTime=sample_time
  reference_h3 : ZeroOrderHold  SampleTime=sample_time
  ua_ref : MATLAB Function  TreatAsAtomicUnit=on
  ua_ref1 : MATLAB Function  TreatAsAtomicUnit=on
  water : Scope  NumInputPorts=6
  zoh{,1..8} (9 alike) : ZeroOrderHold  SampleTime=sample_time
  wires:
  e_h2/1 -> PID h2/1
  plant/2(h2_out) -> water/1, Zero-Order Hold1/1  "h2_cont"
  plant/3(h3_out) -> water/2, Zero-Order Hold/1  "h3_cont"
  plant/5(c3_out) -> Zero-Order Hold2/1, oxygen/1  "c3_cont"
  h3_ref/1(y) -> reference_h3/1
  e_h3/1 -> PID h3/1
  ua_ref/1(y) -> reference_c3/1
  e_c3/1 -> PID c3/1
  Clock/1 -> h3_ref/1(t)
  Clock1/1 -> ua_ref/1(t)
  Water control h3/1 -> control_effort/1, plant/1(ud)  "h3_continuous_control"
  PID c3/1 -> zoh1/1
  Oxygen control c3/1 -> control_effort/2, plant/2(ua)  "c3_continuous_control"
  PID h3/1 -> zoh/1
  Clock2/1 -> ua_ref1/1(t)
  ua_ref1/1(y) -> reference_h2/1
  PID h2/1 -> zoh2/1
  Water control h2/1 -> control_effort/3, plant/3(ur)  "h2_continuous_control"
  Zero-Order Hold1/1 -> e_h2/2
  Zero-Order Hold/1 -> e_h3/2
  Zero-Order Hold2/1 -> e_c3/2
  reference_h2/1 -> e_h2/1, e_h1/1, e_H2/1
  reference_c3/1 -> e_c1/1, e_C3/1, e_c3/1
  reference_h3/1 -> e_h3/1, e_h4/1, e_H3/1
  zoh/1 -> Water control h3/1
  zoh1/1 -> Oxygen control c3/1
  zoh2/1 -> Water control h2/1
  zoh4/1 -> Oxygen control c1/1
  zoh3/1 -> Water control h4/1
  e_H2/1 -> PID H2/1
  Zero-Order Hold5/1 -> e_C3/2
  Water control h1/1 -> control_effort/9, Mux/2  "h2_discrete_control"
  Zero-Order Hold4/1 -> e_H2/2
  PID H3/1 -> zoh3/1
  e_C3/1 -> PID C3/1
  e_H3/1 -> PID H3/1
  Oxygen control c1/1 -> control_effort/8, Mux/1  "c3_discrete_control"
  zoh5/1 -> Water control h1/1
  Zero-Order Hold3/1 -> e_H3/2
  PID H2/1 -> zoh5/1
  Water control h4/1 -> control_effort/7, Mux/3  "h3_discrete_control"
  PID C3/1 -> zoh4/1
  Demux/1 -> water/5, Zero-Order Hold4/1  "h2_disc"
  Demux/2 -> water/6, Zero-Order Hold3/1  "h3_disc"
  Demux/3 -> Zero-Order Hold5/1, oxygen/3  "c3_disc"
  Mux/1 -> Discretized linearized plant/1(In1)
  Discretized linearized plant/1(Out1) -> Demux/1
  zoh7/1 -> Oxygen control c2/1
  e_h1/1 -> control h2/1
  Water control h5/1 -> control_effort/6, Euler/3(ur)  "h2_euler_control"
  Zero-Order Hold7/1 -> e_h1/2
  Zero-Order Hold8/1 -> e_c1/2
  control h3/1 -> zoh6/1
  zoh6/1 -> Water control h6/1
  Zero-Order Hold6/1 -> e_h4/2
  zoh8/1 -> Water control h5/1
  e_h4/1 -> control h3/1
  control h2/1 -> zoh8/1
  Oxygen control c2/1 -> control_effort/5, Euler/2(ua)  "c3_euler_control"
  Water control h6/1 -> control_effort/4, Euler/1(ud)  "h3_euler_control"
  control c3/1 -> zoh7/1
  e_c1/1 -> control c3/1
  Euler/2(h2_out) -> Zero-Order Hold7/1, water/3  "h2_euler"
  Euler/5(c3_out) -> oxygen/2, Zero-Order Hold8/1  "c3_euler"
  Euler/3(h3_out) -> Zero-Order Hold6/1, water/4  "h3_euler"

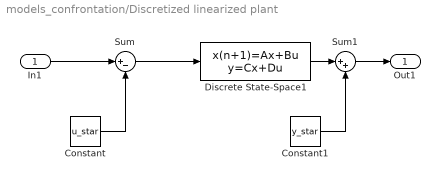
== system models_confrontation/Discretized linearized plant ==
  In1 : Inport
  Constant : Constant  Value=u_star
  Constant1 : Constant  Value=y_star
  Discrete State-Space1 : DiscreteStateSpace  A=A_disc  B=B_disc  C=C_disc  D=D_disc  SampleTime=sample_time
  Sum : Sum  Inputs=|+-
  Sum1 : Sum  Inputs=|++
  Out1 : Outport
  wires:
  In1/1 -> Sum/1
  Constant/1 -> Sum/2
  Sum/1 -> Discrete State-Space1/1
  Discrete State-Space1/1 -> Sum1/1
  Sum1/1 -> Out1/1
  Constant1/1 -> Sum1/2

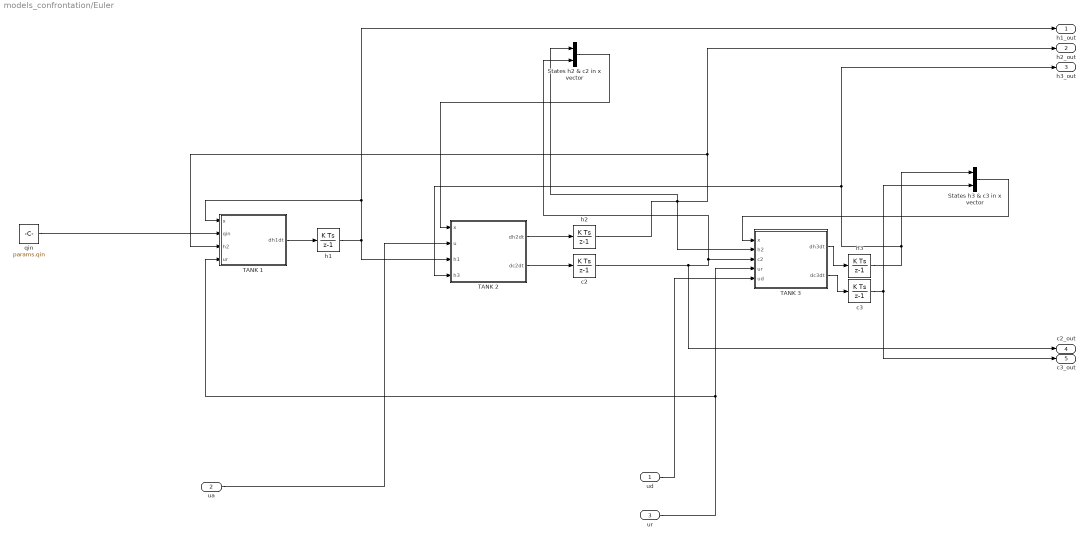
== system models_confrontation/Euler ==
  ud : Inport
  ua : Inport  Port=2
  ur : Inport  Port=3
  States h2 & c2 in x vector : Mux  Inputs=2
  States h3 & c3 in x vector : Mux  Inputs=2
  TANK 1 : MATLAB Function  TreatAsAtomicUnit=on
  TANK 2 : MATLAB Function  TreatAsAtomicUnit=on
  TANK 3 : MATLAB Function  TreatAsAtomicUnit=on
  c2 : DiscreteIntegrator  InitialCondition=c2_init  SampleTime=sample_time  LimitOutput=on  LowerSaturationLimit=0  ICPrevOutput=DiscIntNeverNeededParam  ICPrevScaledInput=DiscIntNeverNeededParam
  c3 : DiscreteIntegrator  InitialCondition=c3_init  SampleTime=sample_time  LimitOutput=on  LowerSaturationLimit=0  ICPrevOutput=DiscIntNeverNeededParam  ICPrevScaledInput=DiscIntNeverNeededParam
  h1 : DiscreteIntegrator  InitialCondition=h1_init  SampleTime=sample_time  LimitOutput=on  LowerSaturationLimit=0  ICPrevOutput=DiscIntNeverNeededParam  ICPrevScaledInput=DiscIntNeverNeededParam
  h2 : DiscreteIntegrator  InitialCondition=h2_init  SampleTime=sample_time  LimitOutput=on  LowerSaturationLimit=0  ICPrevOutput=DiscIntNeverNeededParam  ICPrevScaledInput=DiscIntNeverNeededParam
  h3 : DiscreteIntegrator  InitialCondition=h3_init  SampleTime=sample_time  LimitOutput=on  LowerSaturationLimit=0  ICPrevOutput=DiscIntNeverNeededParam  ICPrevScaledInput=DiscIntNeverNeededParam
  qin : Constant  Value=params.qin
  h1_out : Outport
  h2_out : Outport  Port=2
  h3_out : Outport  Port=3
  c2_out : Outport  Port=4
  c3_out : Outport  Port=5
  wires:
  ua/1 -> TANK 2/2(u)
  ur/1 -> TANK 1/4(ur), TANK 3/4(ur)
  States h2 & c2 in x vector/1 -> TANK 2/1(x)
  TANK 2/2(dc2dt) -> c2/1
  c2/1 -> c2_out/1, States h2 & c2 in x vector/2, TANK 3/3(c2)
  c3/1 -> c3_out/1, States h3 & c3 in x vector/2
  TANK 2/1(dh2dt) -> h2/1
  TANK 1/1(dh1dt) -> h1/1
  TANK 3/1(dh3dt) -> h3/1
  TANK 3/2(dc3dt) -> c3/1
  h3/1 -> h3_out/1, TANK 2/4(h3), States h3 & c3 in x vector/1
  h2/1 -> h2_out/1, TANK 1/3(h2), TANK 3/2(h2), States h2 & c2 in x vector/1
  States h3 & c3 in x vector/1 -> TANK 3/1(x)
  qin/1 -> TANK 1/2(qin)
  h1/1 -> TANK 2/3(h1), h1_out/1, TANK 1/1(x)
  ud/1 -> TANK 3/5(ud)

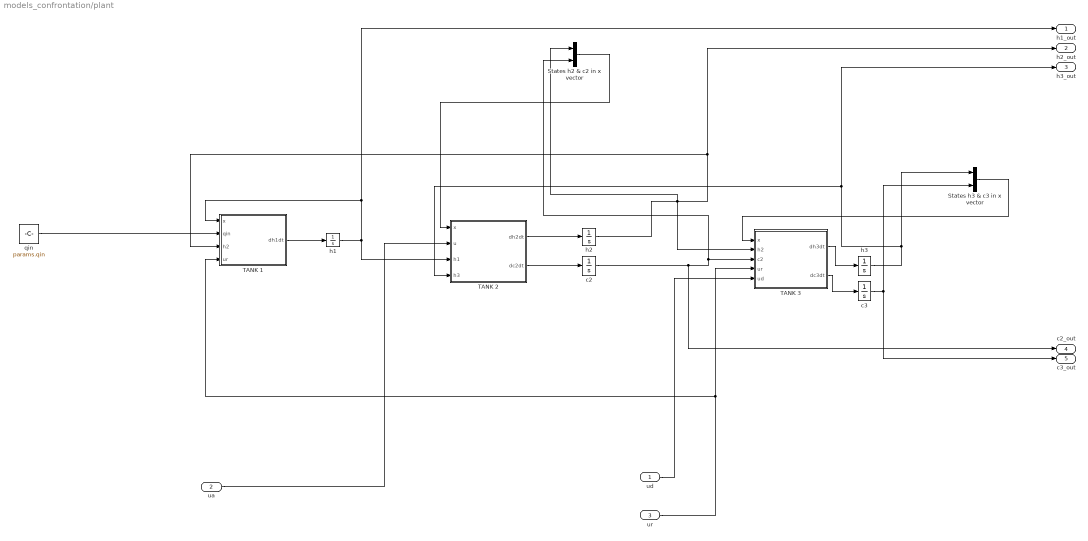
== system models_confrontation/plant ==
  ud : Inport
  ua : Inport  Port=2
  ur : Inport  Port=3
  States h2 & c2 in x vector : Mux  Inputs=2
  States h3 & c3 in x vector : Mux  Inputs=2
  TANK 1 : MATLAB Function  TreatAsAtomicUnit=on
  TANK 2 : MATLAB Function  TreatAsAtomicUnit=on
  TANK 3 : MATLAB Function  TreatAsAtomicUnit=on
  c2 : Integrator  InitialCondition=c2_init  LimitOutput=on  UpperSaturationLimit=8.0  LowerSaturationLimit=0
  c3 : Integrator  InitialCondition=c3_init  LimitOutput=on  LowerSaturationLimit=0
  h1 : Integrator  InitialCondition=h1_init  LimitOutput=on  LowerSaturationLimit=0
  h2 : Integrator  InitialCondition=h2_init  LimitOutput=on  LowerSaturationLimit=0
  h3 : Integrator  InitialCondition=h3_init  LimitOutput=on  LowerSaturationLimit=0
  qin : Constant  Value=params.qin
  h1_out : Outport
  h2_out : Outport  Port=2
  h3_out : Outport  Port=3
  c2_out : Outport  Port=4
  c3_out : Outport  Port=5
  wires:
  ua/1 -> TANK 2/2(u)
  ur/1 -> TANK 1/4(ur), TANK 3/4(ur)
  States h2 & c2 in x vector/1 -> TANK 2/1(x)
  TANK 2/2(dc2dt) -> c2/1
  c2/1 -> c2_out/1, States h2 & c2 in x vector/2, TANK 3/3(c2)
  c3/1 -> c3_out/1, States h3 & c3 in x vector/2
  TANK 2/1(dh2dt) -> h2/1
  TANK 1/1(dh1dt) -> h1/1
  TANK 3/1(dh3dt) -> h3/1
  TANK 3/2(dc3dt) -> c3/1
  h3/1 -> h3_out/1, TANK 2/4(h3), States h3 & c3 in x vector/1
  h2/1 -> h2_out/1, TANK 1/3(h2), TANK 3/2(h2), States h2 & c2 in x vector/1
  States h3 & c3 in x vector/1 -> TANK 3/1(x)
  qin/1 -> TANK 1/2(qin)
  h1/1 -> TANK 2/3(h1), h1_out/1, TANK 1/1(x)
  ud/1 -> TANK 3/5(ud)

== matlab function models_confrontation/plant/TANK 2 ==
  data: x input; u input; dh2dt output size=1; h1 input; h3 input; dc2dt output size=1
function [dh2dt, dc2dt] = tank2(x, u, h1, h3)

%states
h2 = max(x(1), 1e-3);
c2 = max(x(2), 0);
%params
A1 = 1.2;
A2 = 1.0;
cin = 1.0;
k12 = 0.22;
k23 = 0.20;
csat = 8.0;
lambda2 = 0.08;
ka = 0.9;
%input
ua = u;
%flow
q12 = k12 * sqrt(max(h1 - h2, 0));
q23 = k23 * sqrt(max(h2 - h3, 0));
%q23 = min(q23, h2*A2);
eps_h = 1e-2;
%output
dh2dt = (1/A2) * (q12 - q23);
dc2dt = (q12 / (A2 * max(h2, eps_h))) * (cin - c2) + ka * ua * (csat - c2) - lambda2 * c2;
end

== matlab function models_confrontation/plant/TANK 1 ==
  data: x input; qin input; dh1dt output size=1; h2 input; ur input
function dh1dt = tank1(x, qin, h2, ur)
%state
%h1 = max(x, 1e-3);
h1 = x;
%params
A1 = 1.2;
k12 = 0.22;
%input ur
%flow rate
q12 = k12 * sqrt(max(h1 - h2, 0));
%q12 = min(q12, h1*A1);
dh1dt = (1/A1) * (qin + ur - q12);
end

== matlab function models_confrontation/plant/TANK 3 ==
  data: x input; dh3dt output size=1; h2 input; c2 input; dc3dt output size=1; ur input; ud input
function [dh3dt, dc3dt] = tank3(x, h2, c2, ur , ud)

%states
c3 = x(2);
h3 = max(x(1),1e-3);
%params
A2 = 1.0;
A3 = 1.4;
lambda3 = 0.05;
k23 = 0.20;
%flow
q23 = k23 * sqrt(max(h2 - h3, 0));
%q23 = min(q23, h2*A2);
eps_h = 1e-4;
%output
dh3dt = (1/A3) * (q23 - ud - ur);
dc3dt = (q23 / (A3 * max(h3, eps_h))) * (c2 - c3) - lambda3 * c3;

end

== matlab function models_confrontation/ua_ref ==
  data: t input; y output
function y = c3ref(t)

y = 5.50 + 0.70*(1 - exp(-t/40)) + 0.20*sin(2*pi/75 * t);

== matlab function models_confrontation/h3_ref ==
  data: t input; y output
function y = h3ref(t)

y = 0.90 + 0.06*sin(2*pi/90 * t + pi/4);

== matlab function models_confrontation/ua_ref1 ==
  data: t input; y output
function y = h2ref(t)

y = 0.80 + 0.08*sin((2*pi/60)*t);

== matlab function models_confrontation/Euler/TANK 1 ==
  data: x input; qin input; dh1dt output size=1; h2 input; ur input
function dh1dt = tank1(x, qin, h2, ur)
%state
%h1 = max(x, 1e-3);
h1 = x;
%params
A1 = 1.2;
k12 = 0.22;
%input ur
%flow rate
q12 = k12 * sqrt(max(h1 - h2, 0));
%q12 = min(q12, h1*A1);
dh1dt = (1/A1) * (qin + ur - q12);
end

== matlab function models_confrontation/Euler/TANK 2 ==
  data: x input; u input; dh2dt output size=1; h1 input; h3 input; dc2dt output size=1
function [dh2dt, dc2dt] = tank2(x, u, h1, h3)

%states
h2 = max(x(1), 1e-3);
c2 = max(x(2), 0);
%params
A1 = 1.2;
A2 = 1.0;
cin = 1.0;
k12 = 0.22;
k23 = 0.20;
csat = 8.0;
lambda2 = 0.08;
ka = 0.9;
%input
ua = u;
%flow
q12 = k12 * sqrt(max(h1 - h2, 0));
q23 = k23 * sqrt(max(h2 - h3, 0));
%q23 = min(q23, h2*A2);
eps_h = 1e-2;
%output
dh2dt = (1/A2) * (q12 - q23);
dc2dt = (q12 / (A2 * max(h2, eps_h))) * (cin - c2) + ka * ua * (csat - c2) - lambda2 * c2;
end

== matlab function models_confrontation/Euler/TANK 3 ==
  data: x input; dh3dt output size=1; h2 input; c2 input; dc3dt output size=1; ur input; ud input
function [dh3dt, dc3dt] = tank3(x, h2, c2, ur , ud)

%states
c3 = x(2);
h3 = max(x(1),1e-3);
%params
A2 = 1.0;
A3 = 1.4;
lambda3 = 0.05;
k23 = 0.20;
%flow
q23 = k23 * sqrt(max(h2 - h3, 0));
%q23 = min(q23, h2*A2);
eps_h = 1e-4;
%output
dh3dt = (1/A3) * (q23 - ud - ur);
dc3dt = (q23 / (A3 * max(h3, eps_h))) * (c2 - c3) - lambda3 * c3;

end
